simulink model "TServoComnication"  (R2025b)
settings: Solver=ode4  StartTime=0.0  StopTime=inf  FixedStep=0.01  RelTol=1e-3
libraries: ASEToolBox x5, simulink x1
settings Model: Creator=admin  LastModifiedBy=zqhkd
settings DataIOCC: SaveFinalState=on  SaveOutput=off  InspectSignalLogs=on  SaveTime=off
settings OptimizationCC: EnhancedBackFolding=on  PassReuseOutputArgsAs=Individual arguments  ZeroExternalMemoryAtStartup=off  ZeroInternalMemoryAtStartup=off  OptimizeBlockOrder=speed  DifferentSizesBufferReuse=on  OptimizationCustomize=off  EfficientTunableParamExpr=on
settings DebuggingCC: ParameterTunabilityLossMsg=error
settings HardwareCC: ProdBitPerLong=64.0  ProdHWDeviceType=Intel->x86-64 (Linux 64)
settings SFSimCC: MATLABDynamicMemAlloc=off
settings RTWCC: SystemTargetFile=ert.tlc  TemplateMakefile=ert_default_tmf  RetainRTWFile=on  Toolchain=Microsoft Visual C++ 2022 v17.0 | nmake (64-bit Windows)  GPUComputeCapability=3.5  Description=Embedded Coder
settings CodeAppCC: ForceParamTrailComments=on  IgnoreCustomStorageClasses=off  OperatorAnnotations=on  SimulinkDataObjDesc=on  SFDataObjDesc=on  InsertBlockDesc=on
settings ERTTargetCC: InlinedParameterPlacement=Hierarchical  RTWCAPISignals=on  RTWCAPIParams=on  RTWCAPIStates=on  RTWCAPIRootIO=on  ERTCustomFileTemplate=example_file_process.tlc  DynamicArrayContainerType=coder::array  TargetLangStandard=C99 (ISO)  SupportContinuousTime=on

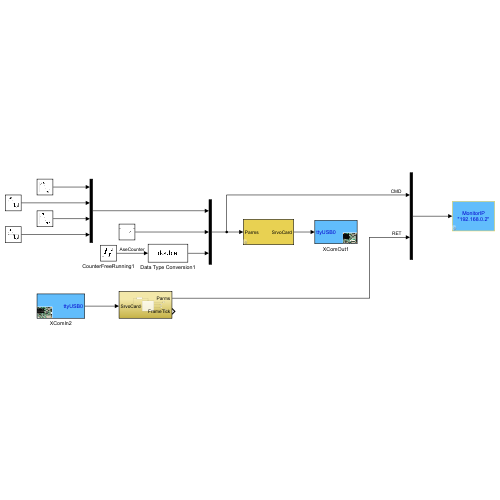
[thumbnail: Simulink's stored preview of the top-level diagram]
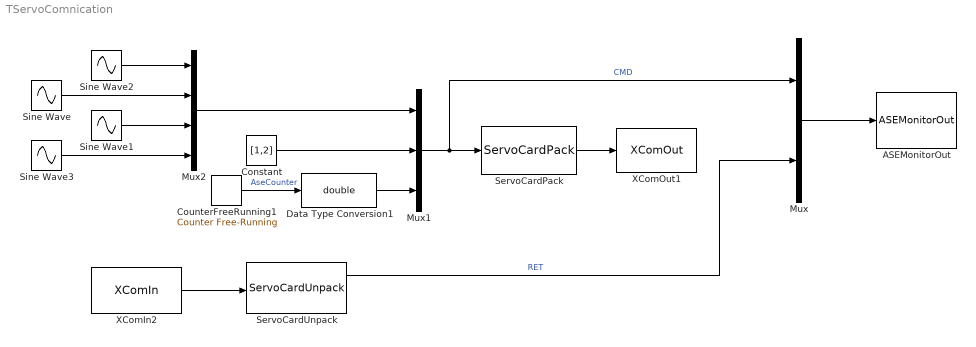
== system TServoComnication ==
  ASEMonitorOut : ASEToolBox/SIMSystemModule/ASEMonitorOut  Tag=ASEMonitorOutTag  g_iVarNum=14  g_iFrameType=10  g_hostIP="\"192.168.0.2\""
      settings: SourceProductName=ASEToolBox
  Constant : Constant  Value=[1,2]
  CounterFreeRunning1 : simulink/Sources/Counter Free-Running  NumBits=32  tsamp=-1
  Data Type Conversion1 : DataTypeConversion  OutDataTypeStr=double  SaturateOnIntegerOverflow=off  RndMeth=Floor
  Mux : Mux  Inputs=2
  Mux1 : Mux  Inputs=[4,2,1]
  Mux2 : Mux
  ServoCardPack : ASEToolBox/ACEModule/ServoCardPack  g_FrameType=80  g_SendId=0
      settings: SourceProductName=ASEToolBox
  ServoCardUnpack : ASEToolBox/ACEModule/ServoCardUnpack  SystemSampleTime=-1  VariantActivationTime=update diagram  EmptyChoice=off  PassThrough=off  PassThroughVariantControl=(default)  EmptyChoiceVariantControl=(default)  AllowFlexibleInterface=on  Latency=0  AutoFrameSizeCalculation=off
      settings: SourceProductName=ASEToolBox
  Sine Wave : Sin  Amplitude=5  Frequency=2*pi*2  SampleTime=0.01
  Sine Wave1 : Sin  Amplitude=10  Frequency=2*pi*2  SampleTime=0.01
  Sine Wave2 : Sin  Frequency=2*pi*2  SampleTime=0.01
  Sine Wave3 : Sin  Amplitude=15  Frequency=2*pi*2  SampleTime=0.01
  XComIn2 : ASEToolBox/COMModule/XComIn  g_serial_select=ttyUSB0  g_baudrate=460800  g_parity=None  g_databit=8  g_stopbit=1  g_data_size=12+7*4  g_sample_time=0.01
      settings: SourceProductName=ASEToolBox
  XComOut1 : ASEToolBox/COMModule/XComOut  g_serial_select=ttyUSB0  g_baudrate=460800  g_parity=None  g_databit=8  g_stopbit=1  g_sample_time=0.01
      settings: SourceProductName=ASEToolBox
  wires:
  Mux/1 -> ASEMonitorOut/1
  ServoCardUnpack/1 -> Mux/2  "RET"
  Constant/1 -> Mux1/2
  Mux1/1 -> ServoCardPack/1, Mux/1  "CMD"
  Mux2/1 -> Mux1/1
  Data Type Conversion1/1 -> Mux1/3
  CounterFreeRunning1/1 -> Data Type Conversion1/1  "AseCounter"
  Sine Wave/1 -> Mux2/2
  Sine Wave1/1 -> Mux2/3
  Sine Wave2/1 -> Mux2/1
  Sine Wave3/1 -> Mux2/4
  XComIn2/1 -> ServoCardUnpack/1
  ServoCardPack/1 -> XComOut1/1
